simulink model "assignment8"  (R2026a)
settings: Solver=VariableStepAuto  StopTime=4
values from neighbouring files (symbols this model uses):
  A = [-4 0; 3 -2]    [assignment.m]
  C = [0 1]    [assignment.m]
  P0 = [0.04 0;0 0.01]    [assignment.m]
  Q = 400    [assignment.m]
settings Model: Creator=saradenti  LastModifiedBy=saradenti

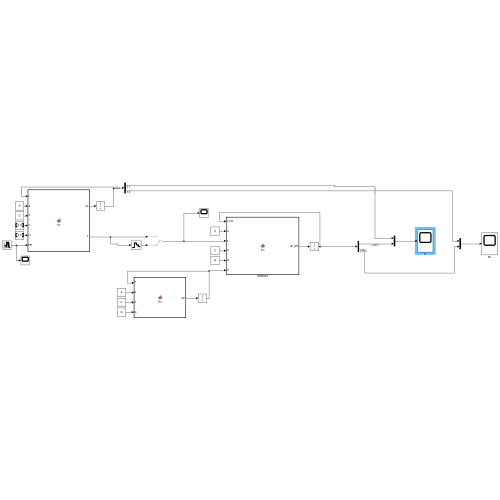
[thumbnail: Simulink's stored preview of the top-level diagram]
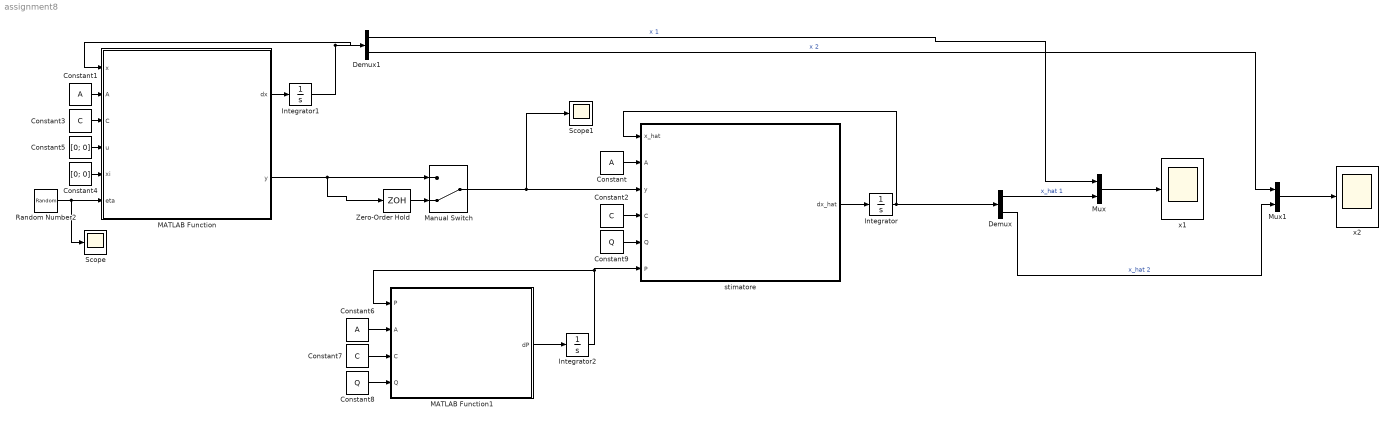
== system assignment8 ==
  Constant : Constant  Value=A
  Constant1 : Constant  Value=A
  Constant2 : Constant  Value=C
  Constant3 : Constant  Value=C
  Constant4 : Constant  Value=[0; 0]
  Constant5 : Constant  Value=[0; 0]
  Constant6 : Constant  Value=A
  Constant7 : Constant  Value=C
  Constant8 : Constant  Value=Q
  Constant9 : Constant  Value=Q
  Demux : Demux  Outputs=2
  Demux1 : Demux  Outputs=2
  Integrator : Integrator  InitialCondition=[0; 0]
  Integrator1 : Integrator  InitialCondition=[0; 0]
  Integrator2 : Integrator  InitialCondition=P0
  MATLAB Function : MATLAB Function  TreatAsAtomicUnit=on
  MATLAB Function1 : MATLAB Function  TreatAsAtomicUnit=on
  Manual Switch : ManualSwitch  CurrentSetting=0
  Mux : Mux  Inputs=2
  Mux1 : Mux  Inputs=2
  Random Number2 : RandomNumber  Variance=0.0025  Seed=12345  SampleTime=0.01
  Scope : Scope
      settings: ActiveDisplayYMinimum=-1  ActiveDisplayYMaximum=1  DataLoggingVariableName=ScopeData5
  Scope1 : Scope
      settings: ActiveDisplayYMinimum=-1  ActiveDisplayYMaximum=1  DataLoggingVariableName=ScopeData6
  Zero-Order Hold : ZeroOrderHold  SampleTime=0.05
  stimatore : MATLAB Function  TreatAsAtomicUnit=on
  x1 : Scope
      settings: ActiveDisplayYMinimum=-0.0071852041866489755  ActiveDisplayYMaximum=0.0054847122097662964
  x2 : Scope
      settings: ActiveDisplayYMinimum=-0.093691287455379774  ActiveDisplayYMaximum=0.051346858636782261
  wires:
  stimatore/1(dx_hat) -> Integrator/1
  Constant/1 -> stimatore/2(A)
  Random Number2/1 -> Scope/1, MATLAB Function/6(eta)
  Constant2/1 -> stimatore/4(C)
  MATLAB Function/1(dx) -> Integrator1/1
  Integrator1/1 -> MATLAB Function/1(x), Demux1/1
  Constant1/1 -> MATLAB Function/2(A)
  Constant3/1 -> MATLAB Function/3(C)
  Constant4/1 -> MATLAB Function/5(xi)
  MATLAB Function/2(y) -> Manual Switch/1, Zero-Order Hold/1
  Constant5/1 -> MATLAB Function/4(u)
  MATLAB Function1/1(dP) -> Integrator2/1
  Integrator2/1 -> stimatore/6(P), MATLAB Function1/1(P)
  Constant6/1 -> MATLAB Function1/2(A)
  Constant7/1 -> MATLAB Function1/3(C)
  Constant8/1 -> MATLAB Function1/4(Q)
  Constant9/1 -> stimatore/5(Q)
  Integrator/1 -> Demux/1, stimatore/1(x_hat)
  Mux/1 -> x1/1
  Demux/1 -> Mux/2  "x_hat 1"
  Demux/2 -> Mux1/2  "x_hat 2"
  Demux1/1 -> Mux/1  "x 1"
  Demux1/2 -> Mux1/1  "x 2"
  Mux1/1 -> x2/1
  Manual Switch/1 -> Scope1/1, stimatore/3(y)
  Zero-Order Hold/1 -> Manual Switch/2

== matlab function assignment8/MATLAB Function ==
  data: x input; A input; C input; dx output; u input; y output; xi input; eta input
function [dx, y] = fcn(x, A, C, u, xi, eta)


    x  = reshape(x,  2, 1);
    C  = reshape(C,  1, 2);
    u  = reshape(u,  2, 1);
    xi = reshape(xi, 2, 1);

    dx = A * x + u + xi;
    y = C* x + eta;

== matlab function assignment8/stimatore ==
  data: x_hat input; A input; dx_hat output; y input; C input; Q input; P input
function dx_hat = fcn(x_hat, A, y, C,Q, P)

x_hat = reshape(x_hat, 2, 1);
C     = reshape(C, 1, 2);
P     = reshape(P, 2, 2);

    K = P * transpose(C) * Q;
    dx_hat = A * x_hat + K * (y - C * x_hat);

== matlab function assignment8/MATLAB Function1 ==
  data: P input; A input; dP output; C input; Q input
function dP = fcn(P, A, C, Q)

P = reshape(P, 2, 2);
C = reshape(C, 1, 2);

    dP = A * P + P * transpose(A) - P * transpose(C) * Q * C * P;
